simulink model "model_23b"  (R2023b)
settings: Solver=ode45  StartTime=TSPAN(1)  StopTime=TSPAN(2)  MaxStep=MaxStep  RelTol=RelTol  AbsTol=AbsTol
values from neighbouring files (symbols this model uses):
  cal_V0_ini = 0    [init.m]
  dim_xp = numel(xp_0)    [init.m]
  JSPAN = [0 30*TSPAN(2)]    [init.m]
  parameters = struct()    [init.m]
  TSPAN = [0 300]    [init.m]
  xc_0 = [chi_0;theta_0]    [init.m]
  xp_0 = [p_0;q_0;v_0;o_0]    [init.m]
libraries: HyEQ_Library x6
(part 1 of 2)
settings Model: Creator=score  LastModifiedBy=zxz
settings DataIOCC: SaveFormat=Array  ReturnWorkspaceOutputs=off

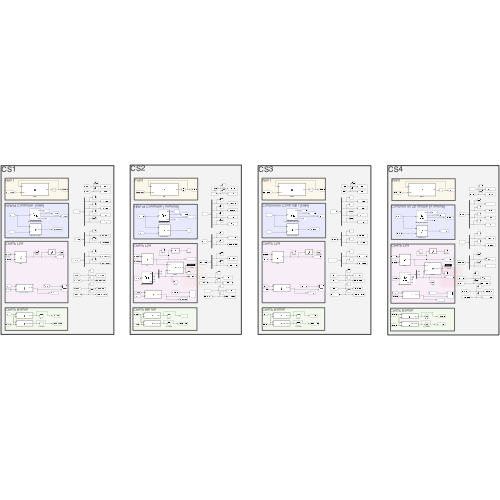
[thumbnail: Simulink's stored preview of the top-level diagram]
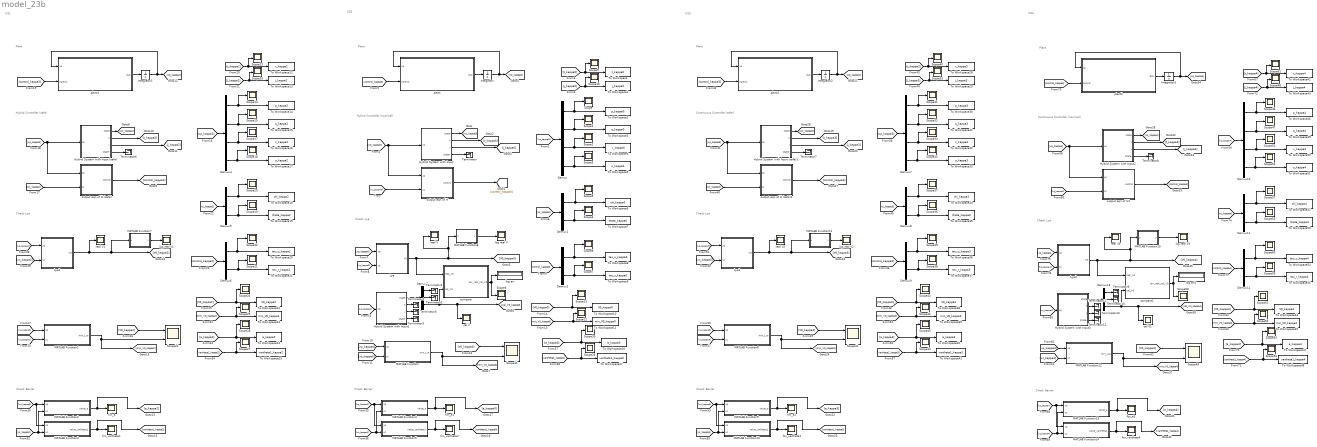
== system model_23b ==
  note: CS2
  note: CS1
  note: Check Barrier
  note: Check Lya
  note: Plant
  note: Hybrid Controller (nominal)
  note: Plant
  note: Hybrid Controller (safe)
  note: Check Lya
  note: Check Barrier
  note: CS3
  note: Continuous Controller (safe)
  note: Check Barrier
  note: Check Lya
  note: Plant
  note: CS4
  note: Check Barrier
  note: Plant
  note: Continuous Controller (nominal)
  note: Check Lya
  Demux{,4,7,10} (4 alike) : Demux  Outputs=[2;2;2;1]
  Demux{1,5,8,11} (4 alike) : Demux  Outputs=[2;1]
  Demux{2,6,9,12} (4 alike) : Demux  Outputs=[1;1]
  Demux13 : Demux  Outputs=[2;1;1]
  Demux3 : Demux  Outputs=[2;1;1]
  Hybrid System with Input : Subsystem  LoadFcn=set_param(gcb,'LinkStatus','none')  mask(Hybrid System with Inputs){x0=xc_0, input_dim=dim_xp, parameters=parameters, T=TSPAN(2), J=JSPAN(2), rule=Flow}
      mask prompts: x0 "Initial Condition (column vector)"; input_dim "Input Dimension (positive integer)"; T "Flow Horizon (nonnegative real)"; J "Jump Horizon (nonnegative integer)"; rule "Flow/Jump Priorty Rule"
      mask help:
      | To modify (f, g, C, D) for this block, "Look inside" the block mask by either clicking the down arrow in the lower-left corner or selecting "Mask" > "Look Under Mask" from the context menu.
      |
      | For instructions how to use this block, see the
      mask init:
      | state_dim = numel(x0);
      settings: CopyFcn=|
      | set_param(gcb,'LinkStatus','none'),
      | set_param(gcs, 'MaxStep', 'MaxStep', 'RelTol', 'RelTol','StopTime', 'T')
      mask Help:
      | To modify (f, g, C, D) for this block, "Look inside" the block mask by either clicking the down arrow in the lower-left corner or selecting "Mask" > "Look Under Mask" from the context menu.
      | 
      | The value given in the 'parameters' field is passed as the last input argument for f, g, C, and D. Any MATLAB object can be used, but we recommend using a struct. For example, in the initialization script, a parameters struct can be defined as followed.
      |   parameters = struct();
      |   parameters.A = eye(2);
      |   parameters.B = [1; 0];
      | 
      | The output "x-" is the state output delayed by one integration step. Use this output to break algebraic loops.
      mask TypeOptions x0: Integrator System/x0
      mask TypeOptions T: Integrator System/T
      mask TypeOptions J: Integrator System/J
      mask TypeOptions rule: Jump | Flow | Random
      mask DialogControl Control2 Prompt: Introduction to the HyEQ Simulink-based Library
      mask DialogControl Control2 Callback: hybrid.internal.openHelp('Help_SimulinkLibrary')
      mask DialogControl Container3 Prompt: System Configuration
      mask DialogControl Container2 Prompt: Solver Options
      mask Display:
      | image('Hcal.jpg')
      | port_label('output', 1, 'state')
      | port_label('output', 2, 't')
      | port_label('output', 3, 'j')
      | port_label('output', 4, 'state^-','texmode', 'on')
      | port_label('input', 1, 'xp')
  Hybrid System with Input (safe) : Subsystem  LoadFcn=set_param(gcb,'LinkStatus','none')  mask(Hybrid System with Inputs){x0=xc_0, input_dim=dim_xp, parameters=parameters, T=TSPAN(2), J=JSPAN(2), rule=Flow}
      mask prompts: x0 "Initial Condition (column vector)"; input_dim "Input Dimension (positive integer)"; T "Flow Horizon (nonnegative real)"; J "Jump Horizon (nonnegative integer)"; rule "Flow/Jump Priorty Rule"
      mask help:
      | To modify (f, g, C, D) for this block, "Look inside" the block mask by either clicking the down arrow in the lower-left corner or selecting "Mask" > "Look Under Mask" from the context menu.
      |
      | For instructions how to use this block, see the
      mask init:
      | state_dim = numel(x0);
      settings: CopyFcn=|
      | set_param(gcb,'LinkStatus','none'),
      | set_param(gcs, 'MaxStep', 'MaxStep', 'RelTol', 'RelTol','StopTime', 'T')
      mask Help:
      | To modify (f, g, C, D) for this block, "Look inside" the block mask by either clicking the down arrow in the lower-left corner or selecting "Mask" > "Look Under Mask" from the context menu.
      | 
      | The value given in the 'parameters' field is passed as the last input argument for f, g, C, and D. Any MATLAB object can be used, but we recommend using a struct. For example, in the initialization script, a parameters struct can be defined as followed.
      |   parameters = struct();
      |   parameters.A = eye(2);
      |   parameters.B = [1; 0];
      | 
      | The output "x-" is the state output delayed by one integration step. Use this output to break algebraic loops.
      mask TypeOptions x0: Integrator System/x0
      mask TypeOptions T: Integrator System/T
      mask TypeOptions J: Integrator System/J
      mask TypeOptions rule: Jump | Flow | Random
      mask DialogControl Control2 Prompt: Introduction to the HyEQ Simulink-based Library
      mask DialogControl Control2 Callback: hybrid.internal.openHelp('Help_SimulinkLibrary')
      mask DialogControl Container3 Prompt: System Configuration
      mask DialogControl Container2 Prompt: Solver Options
      mask Display:
      | image('Hcal.jpg')
      | port_label('output', 1, 'state')
      | port_label('output', 2, 't')
      | port_label('output', 3, 'j')
      | port_label('output', 4, 'state^-','texmode', 'on')
      | port_label('input', 1, 'xp')
  Hybrid System with Input (safe)1 : Subsystem  LoadFcn=set_param(gcb,'LinkStatus','none')  mask(Hybrid System with Inputs){x0=xc_0, input_dim=dim_xp, parameters=parameters, T=TSPAN(2), J=JSPAN(2), rule=Flow}
      mask prompts: x0 "Initial Condition (column vector)"; input_dim "Input Dimension (positive integer)"; T "Flow Horizon (nonnegative real)"; J "Jump Horizon (nonnegative integer)"; rule "Flow/Jump Priorty Rule"
      mask help:
      | To modify (f, g, C, D) for this block, "Look inside" the block mask by either clicking the down arrow in the lower-left corner or selecting "Mask" > "Look Under Mask" from the context menu.
      |
      | For instructions how to use this block, see the
      mask init:
      | state_dim = numel(x0);
      settings: CopyFcn=|
      | set_param(gcb,'LinkStatus','none'),
      | set_param(gcs, 'MaxStep', 'MaxStep', 'RelTol', 'RelTol','StopTime', 'T')
      mask Help:
      | To modify (f, g, C, D) for this block, "Look inside" the block mask by either clicking the down arrow in the lower-left corner or selecting "Mask" > "Look Under Mask" from the context menu.
      | 
      | The value given in the 'parameters' field is passed as the last input argument for f, g, C, and D. Any MATLAB object can be used, but we recommend using a struct. For example, in the initialization script, a parameters struct can be defined as followed.
      |   parameters = struct();
      |   parameters.A = eye(2);
      |   parameters.B = [1; 0];
      | 
      | The output "x-" is the state output delayed by one integration step. Use this output to break algebraic loops.
      mask TypeOptions x0: Integrator System/x0
      mask TypeOptions T: Integrator System/T
      mask TypeOptions J: Integrator System/J
      mask TypeOptions rule: Jump | Flow | Random
      mask DialogControl Control2 Prompt: Introduction to the HyEQ Simulink-based Library
      mask DialogControl Control2 Callback: hybrid.internal.openHelp('Help_SimulinkLibrary')
      mask DialogControl Container3 Prompt: System Configuration
      mask DialogControl Container2 Prompt: Solver Options
      mask Display:
      | image('Hcal.jpg')
      | port_label('output', 1, 'state')
      | port_label('output', 2, 't')
      | port_label('output', 3, 'j')
      | port_label('output', 4, 'state^-','texmode', 'on')
      | port_label('input', 1, 'xp')
  Hybrid System with Input1 : Subsystem  LoadFcn=set_param(gcb,'LinkStatus','none')  mask(Hybrid System with Inputs){x0=[xc_0;cal_V0_ini], input_dim=dim_xp, parameters=parameters, T=TSPAN(2), J=JSPAN(2), rule=Flow}
      mask prompts: x0 "Initial Condition (column vector)"; input_dim "Input Dimension (positive integer)"; T "Flow Horizon (nonnegative real)"; J "Jump Horizon (nonnegative integer)"; rule "Flow/Jump Priorty Rule"
      mask help:
      | To modify (f, g, C, D) for this block, "Look inside" the block mask by either clicking the down arrow in the lower-left corner or selecting "Mask" > "Look Under Mask" from the context menu.
      |
      | For instructions how to use this block, see the
      mask init:
      | state_dim = numel(x0);
      settings: CopyFcn=|
      | set_param(gcb,'LinkStatus','none'),
      | set_param(gcs, 'MaxStep', 'MaxStep', 'RelTol', 'RelTol','StopTime', 'T')
      mask Help:
      | To modify (f, g, C, D) for this block, "Look inside" the block mask by either clicking the down arrow in the lower-left corner or selecting "Mask" > "Look Under Mask" from the context menu.
      | 
      | The value given in the 'parameters' field is passed as the last input argument for f, g, C, and D. Any MATLAB object can be used, but we recommend using a struct. For example, in the initialization script, a parameters struct can be defined as followed.
      |   parameters = struct();
      |   parameters.A = eye(2);
      |   parameters.B = [1; 0];
      | 
      | The output "x-" is the state output delayed by one integration step. Use this output to break algebraic loops.
      mask TypeOptions x0: Integrator System/x0
      mask TypeOptions T: Integrator System/T
      mask TypeOptions J: Integrator System/J
      mask TypeOptions rule: Jump | Flow | Random
      mask DialogControl Control2 Prompt: Introduction to the HyEQ Simulink-based Library
      mask DialogControl Control2 Callback: hybrid.internal.openHelp('Help_SimulinkLibrary')
      mask DialogControl Container3 Prompt: System Configuration
      mask DialogControl Container2 Prompt: Solver Options
      mask Display:
      | image('Hcal.jpg')
      | port_label('output', 1, 'state')
      | port_label('output', 2, 't')
      | port_label('output', 3, 'j')
      | port_label('output', 4, 'state^-','texmode', 'on')
      | port_label('input', 1, 'xp')
  Hybrid System with Input2 : Subsystem  LoadFcn=set_param(gcb,'LinkStatus','none')  mask(Hybrid System with Inputs){x0=xc_0, input_dim=dim_xp, parameters=parameters, T=TSPAN(2), J=JSPAN(2), rule=Flow}
      mask prompts: x0 "Initial Condition (column vector)"; input_dim "Input Dimension (positive integer)"; T "Flow Horizon (nonnegative real)"; J "Jump Horizon (nonnegative integer)"; rule "Flow/Jump Priorty Rule"
      mask help:
      | To modify (f, g, C, D) for this block, "Look inside" the block mask by either clicking the down arrow in the lower-left corner or selecting "Mask" > "Look Under Mask" from the context menu.
      |
      | For instructions how to use this block, see the
      mask init:
      | state_dim = numel(x0);
      settings: CopyFcn=|
      | set_param(gcb,'LinkStatus','none'),
      | set_param(gcs, 'MaxStep', 'MaxStep', 'RelTol', 'RelTol','StopTime', 'T')
      mask Help:
      | To modify (f, g, C, D) for this block, "Look inside" the block mask by either clicking the down arrow in the lower-left corner or selecting "Mask" > "Look Under Mask" from the context menu.
      | 
      | The value given in the 'parameters' field is passed as the last input argument for f, g, C, and D. Any MATLAB object can be used, but we recommend using a struct. For example, in the initialization script, a parameters struct can be defined as followed.
      |   parameters = struct();
      |   parameters.A = eye(2);
      |   parameters.B = [1; 0];
      | 
      | The output "x-" is the state output delayed by one integration step. Use this output to break algebraic loops.
      mask TypeOptions x0: Integrator System/x0
      mask TypeOptions T: Integrator System/T
      mask TypeOptions J: Integrator System/J
      mask TypeOptions rule: Jump | Flow | Random
      mask DialogControl Control2 Prompt: Introduction to the HyEQ Simulink-based Library
      mask DialogControl Control2 Callback: hybrid.internal.openHelp('Help_SimulinkLibrary')
      mask DialogControl Container3 Prompt: System Configuration
      mask DialogControl Container2 Prompt: Solver Options
      mask Display:
      | image('Hcal.jpg')
      | port_label('output', 1, 'state')
      | port_label('output', 2, 't')
      | port_label('output', 3, 'j')
      | port_label('output', 4, 'state^-','texmode', 'on')
      | port_label('input', 1, 'xp')
  Hybrid System with Input3 : Subsystem  LoadFcn=set_param(gcb,'LinkStatus','none')  mask(Hybrid System with Inputs){x0=[xc_0;cal_V0_ini], input_dim=dim_xp, parameters=parameters, T=TSPAN(2), J=JSPAN(2), rule=Flow}
      mask prompts: x0 "Initial Condition (column vector)"; input_dim "Input Dimension (positive integer)"; T "Flow Horizon (nonnegative real)"; J "Jump Horizon (nonnegative integer)"; rule "Flow/Jump Priorty Rule"
      mask help:
      | To modify (f, g, C, D) for this block, "Look inside" the block mask by either clicking the down arrow in the lower-left corner or selecting "Mask" > "Look Under Mask" from the context menu.
      |
      | For instructions how to use this block, see the
      mask init:
      | state_dim = numel(x0);
      settings: CopyFcn=|
      | set_param(gcb,'LinkStatus','none'),
      | set_param(gcs, 'MaxStep', 'MaxStep', 'RelTol', 'RelTol','StopTime', 'T')
      mask Help:
      | To modify (f, g, C, D) for this block, "Look inside" the block mask by either clicking the down arrow in the lower-left corner or selecting "Mask" > "Look Under Mask" from the context menu.
      | 
      | The value given in the 'parameters' field is passed as the last input argument for f, g, C, and D. Any MATLAB object can be used, but we recommend using a struct. For example, in the initialization script, a parameters struct can be defined as followed.
      |   parameters = struct();
      |   parameters.A = eye(2);
      |   parameters.B = [1; 0];
      | 
      | The output "x-" is the state output delayed by one integration step. Use this output to break algebraic loops.
      mask TypeOptions x0: Integrator System/x0
      mask TypeOptions T: Integrator System/T
      mask TypeOptions J: Integrator System/J
      mask TypeOptions rule: Jump | Flow | Random
      mask DialogControl Control2 Prompt: Introduction to the HyEQ Simulink-based Library
      mask DialogControl Control2 Callback: hybrid.internal.openHelp('Help_SimulinkLibrary')
      mask DialogControl Container3 Prompt: System Configuration
      mask DialogControl Container2 Prompt: Solver Options
      mask Display:
      | image('Hcal.jpg')
      | port_label('output', 1, 'state')
      | port_label('output', 2, 't')
      | port_label('output', 3, 'j')
      | port_label('output', 4, 'state^-','texmode', 'on')
      | port_label('input', 1, 'xp')
  Integrator{,1..3} (4 alike) : Integrator  InitialCondition=xp_0
  Lya : MATLAB Function  TreatAsAtomicUnit=on
  Lya1 : MATLAB Function  TreatAsAtomicUnit=on
  Lya2 : MATLAB Function  TreatAsAtomicUnit=on
  Lya3 : MATLAB Function  TreatAsAtomicUnit=on
  MATLAB Function : MATLAB Function  TreatAsAtomicUnit=on
  MATLAB Function1 : MATLAB Function  TreatAsAtomicUnit=on
  MATLAB Function10 : MATLAB Function  TreatAsAtomicUnit=on
  MATLAB Function11 : MATLAB Function  TreatAsAtomicUnit=on
  MATLAB Function12 : MATLAB Function  TreatAsAtomicUnit=on
  MATLAB Function13 : MATLAB Function  TreatAsAtomicUnit=on
  MATLAB Function14 : MATLAB Function  TreatAsAtomicUnit=on
  MATLAB Function15 : MATLAB Function  TreatAsAtomicUnit=on
  MATLAB Function2 : MATLAB Function  TreatAsAtomicUnit=on
  MATLAB Function3 : MATLAB Function  TreatAsAtomicUnit=on
  MATLAB Function4 : MATLAB Function  TreatAsAtomicUnit=on
  MATLAB Function5 : MATLAB Function  TreatAsAtomicUnit=on
  MATLAB Function6 : MATLAB Function  TreatAsAtomicUnit=on
  MATLAB Function7 : MATLAB Function  TreatAsAtomicUnit=on
  MATLAB Function8 : MATLAB Function  TreatAsAtomicUnit=on
  MATLAB Function9 : MATLAB Function  TreatAsAtomicUnit=on
  Scope{,1..10,12..23,25..40,42..48,50..61} (58 alike) : Scope
  Scope{11,24,41,49} (4 alike) : Scope  NumInputPorts=2
  Terminator{,1..13} (14 alike) : Terminator
  To Workspace : ToWorkspace  VariableName=t_kappa0  SaveFormat=Structure  SampleTime=-1
      settings: Save2DSignal=2-D array (concatenate along first dimension)
  To Workspace1 : ToWorkspace  VariableName=j_kappa0  SaveFormat=Structure  SampleTime=-1
      settings: Save2DSignal=2-D array (concatenate along first dimension)
  To Workspace10 : ToWorkspace  VariableName=V0_kappa0  SaveFormat=Structure  SampleTime=-1
      settings: Save2DSignal=2-D array (concatenate along first dimension)
  To Workspace11 : ToWorkspace  VariableName=min_V0_kappa0  SaveFormat=Structure  SampleTime=-1
      settings: Save2DSignal=2-D array (concatenate along first dimension)
  To Workspace12 : ToWorkspace  VariableName=t_kappa2  SaveFormat=Structure  SampleTime=-1
      settings: Save2DSignal=2-D array (concatenate along first dimension)
  To Workspace13 : ToWorkspace  VariableName=j_kappa2  SaveFormat=Structure  SampleTime=-1
      settings: Save2DSignal=2-D array (concatenate along first dimension)
  To Workspace14 : ToWorkspace  VariableName=p_kappa2  SaveFormat=Structure  SampleTime=-1
      settings: Save2DSignal=2-D array (concatenate along first dimension)
  To Workspace15 : ToWorkspace  VariableName=q_kappa2  SaveFormat=Structure  SampleTime=-1
      settings: Save2DSignal=2-D array (concatenate along first dimension)
  To Workspace16 : ToWorkspace  VariableName=v_kappa2  SaveFormat=Structure  SampleTime=-1
      settings: Save2DSignal=2-D array (concatenate along first dimension)
  To Workspace17 : ToWorkspace  VariableName=o_kappa2  SaveFormat=Structure  SampleTime=-1
      settings: Save2DSignal=2-D array (concatenate along first dimension)
  To Workspace18 : ToWorkspace  VariableName=chi_kappa2  SaveFormat=Structure  SampleTime=-1
      settings: Save2DSignal=2-D array (concatenate along first dimension)
  To Workspace19 : ToWorkspace  VariableName=theta_kappa2  SaveFormat=Structure  SampleTime=-1
      settings: Save2DSignal=2-D array (concatenate along first dimension)
  To Workspace2 : ToWorkspace  VariableName=p_kappa0  SaveFormat=Structure  SampleTime=-1
      settings: Save2DSignal=2-D array (concatenate along first dimension)
  To Workspace20 : ToWorkspace  VariableName=tau_u_kappa2  SaveFormat=Structure  SampleTime=-1
      settings: Save2DSignal=2-D array (concatenate along first dimension)
  To Workspace21 : ToWorkspace  VariableName=tau_r_kappa2  SaveFormat=Structure  SampleTime=-1
      settings: Save2DSignal=2-D array (concatenate along first dimension)
  To Workspace22 : ToWorkspace  VariableName=V0_kappa2  SaveFormat=Structure  SampleTime=-1
      settings: Save2DSignal=2-D array (concatenate along first dimension)
  To Workspace23 : ToWorkspace  VariableName=min_V0_kappa2  SaveFormat=Structure  SampleTime=-1
      settings: Save2DSignal=2-D array (concatenate along first dimension)
  To Workspace24 : ToWorkspace  VariableName=a_kappa2  SaveFormat=Structure  SampleTime=-1
      settings: Save2DSignal=2-D array (concatenate along first dimension)
  To Workspace25 : ToWorkspace  VariableName=vartheta1_kappa2  SaveFormat=Structure  SampleTime=-1
      settings: Save2DSignal=2-D array (concatenate along first dimension)
  To Workspace26 : ToWorkspace  VariableName=a_kappa0  SaveFormat=Structure  SampleTime=-1
      settings: Save2DSignal=2-D array (concatenate along first dimension)
  To Workspace27 : ToWorkspace  VariableName=vartheta1_kappa0  SaveFormat=Structure  SampleTime=-1
      settings: Save2DSignal=2-D array (concatenate along first dimension)
  To Workspace28 : ToWorkspace  VariableName=t_kappa3  SaveFormat=Structure  SampleTime=-1
      settings: Save2DSignal=2-D array (concatenate along first dimension)
  To Workspace29 : ToWorkspace  VariableName=j_kappa3  SaveFormat=Structure  SampleTime=-1
      settings: Save2DSignal=2-D array (concatenate along first dimension)
  To Workspace3 : ToWorkspace  VariableName=q_kappa0  SaveFormat=Structure  SampleTime=-1
      settings: Save2DSignal=2-D array (concatenate along first dimension)
  To Workspace30 : ToWorkspace  VariableName=p_kappa3  SaveFormat=Structure  SampleTime=-1
      settings: Save2DSignal=2-D array (concatenate along first dimension)
  To Workspace31 : ToWorkspace  VariableName=q_kappa3  SaveFormat=Structure  SampleTime=-1
      settings: Save2DSignal=2-D array (concatenate along first dimension)
  To Workspace32 : ToWorkspace  VariableName=v_kappa3  SaveFormat=Structure  SampleTime=-1
      settings: Save2DSignal=2-D array (concatenate along first dimension)
  To Workspace33 : ToWorkspace  VariableName=o_kappa3  SaveFormat=Structure  SampleTime=-1
      settings: Save2DSignal=2-D array (concatenate along first dimension)
  To Workspace34 : ToWorkspace  VariableName=chi_kappa3  SaveFormat=Structure  SampleTime=-1
      settings: Save2DSignal=2-D array (concatenate along first dimension)
  To Workspace35 : ToWorkspace  VariableName=theta_kappa3  SaveFormat=Structure  SampleTime=-1
      settings: Save2DSignal=2-D array (concatenate along first dimension)
  To Workspace36 : ToWorkspace  VariableName=tau_u_kappa3  SaveFormat=Structure  SampleTime=-1
      settings: Save2DSignal=2-D array (concatenate along first dimension)
  To Workspace37 : ToWorkspace  VariableName=tau_r_kappa3  SaveFormat=Structure  SampleTime=-1
      settings: Save2DSignal=2-D array (concatenate along first dimension)
  To Workspace38 : ToWorkspace  VariableName=V0_kappa3  SaveFormat=Structure  SampleTime=-1
      settings: Save2DSignal=2-D array (concatenate along first dimension)
  To Workspace39 : ToWorkspace  VariableName=min_V0_kappa3  SaveFormat=Structure  SampleTime=-1
      settings: Save2DSignal=2-D array (concatenate along first dimension)
  To Workspace4 : ToWorkspace  VariableName=v_kappa0  SaveFormat=Structure  SampleTime=-1
      settings: Save2DSignal=2-D array (concatenate along first dimension)
  To Workspace40 : ToWorkspace  VariableName=a_kappa3  SaveFormat=Structure  SampleTime=-1
      settings: Save2DSignal=2-D array (concatenate along first dimension)
  To Workspace41 : ToWorkspace  VariableName=vartheta1_kappa3  SaveFormat=Structure  SampleTime=-1
      settings: Save2DSignal=2-D array (concatenate along first dimension)
  To Workspace42 : ToWorkspace  VariableName=t_kappa4  SaveFormat=Structure  SampleTime=-1
      settings: Save2DSignal=2-D array (concatenate along first dimension)
  To Workspace43 : ToWorkspace  VariableName=j_kappa4  SaveFormat=Structure  SampleTime=-1
      settings: Save2DSignal=2-D array (concatenate along first dimension)
  To Workspace44 : ToWorkspace  VariableName=V0_kappa4  SaveFormat=Structure  SampleTime=-1
      settings: Save2DSignal=2-D array (concatenate along first dimension)
  To Workspace45 : ToWorkspace  VariableName=min_V0_kappa4  SaveFormat=Structure  SampleTime=-1
      settings: Save2DSignal=2-D array (concatenate along first dimension)
  To Workspace46 : ToWorkspace  VariableName=p_kappa4  SaveFormat=Structure  SampleTime=-1
      settings: Save2DSignal=2-D array (concatenate along first dimension)
  To Workspace47 : ToWorkspace  VariableName=a_kappa4  SaveFormat=Structure  SampleTime=-1
      settings: Save2DSignal=2-D array (concatenate along first dimension)
  To Workspace48 : ToWorkspace  VariableName=vartheta1_kappa4  SaveFormat=Structure  SampleTime=-1
      settings: Save2DSignal=2-D array (concatenate along first dimension)
  To Workspace49 : ToWorkspace  VariableName=q_kappa4  SaveFormat=Structure  SampleTime=-1
      settings: Save2DSignal=2-D array (concatenate along first dimension)
  To Workspace5 : ToWorkspace  VariableName=o_kappa0  SaveFormat=Structure  SampleTime=-1
      settings: Save2DSignal=2-D array (concatenate along first dimension)
  To Workspace50 : ToWorkspace  VariableName=v_kappa4  SaveFormat=Structure  SampleTime=-1
      settings: Save2DSignal=2-D array (concatenate along first dimension)
  To Workspace51 : ToWorkspace  VariableName=o_kappa4  SaveFormat=Structure  SampleTime=-1
      settings: Save2DSignal=2-D array (concatenate along first dimension)
  To Workspace52 : ToWorkspace  VariableName=chi_kappa4  SaveFormat=Structure  SampleTime=-1
      settings: Save2DSignal=2-D array (concatenate along first dimension)
  To Workspace53 : ToWorkspace  VariableName=theta_kappa4  SaveFormat=Structure  SampleTime=-1
      settings: Save2DSignal=2-D array (concatenate along first dimension)
  To Workspace54 : ToWorkspace  VariableName=tau_u_kappa4  SaveFormat=Structure  SampleTime=-1
      settings: Save2DSignal=2-D array (concatenate along first dimension)
  To Workspace55 : ToWorkspace  VariableName=tau_r_kappa4  SaveFormat=Structure  SampleTime=-1
      settings: Save2DSignal=2-D array (concatenate along first dimension)
  To Workspace6 : ToWorkspace  VariableName=chi_kappa0  SaveFormat=Structure  SampleTime=-1
      settings: Save2DSignal=2-D array (concatenate along first dimension)
  To Workspace7 : ToWorkspace  VariableName=theta_kappa0  SaveFormat=Structure  SampleTime=-1
      settings: Save2DSignal=2-D array (concatenate along first dimension)
  To Workspace8 : ToWorkspace  VariableName=tau_u_kappa0  SaveFormat=Structure  SampleTime=-1
      settings: Save2DSignal=2-D array (concatenate along first dimension)
  To Workspace9 : ToWorkspace  VariableName=tau_r_kappa0  SaveFormat=Structure  SampleTime=-1
      settings: Save2DSignal=2-D array (concatenate along first dimension)
  cal V : Scope
  cal V1 : Scope
  compare : MATLAB Function  TreatAsAtomicUnit=on
  compare1 : MATLAB Function  TreatAsAtomicUnit=on
  fcn_a{,1..3} (4 alike) : Scope
  fcn_vartheta{1..4} (4 alike) : Scope
  log err : Display
  log err1 : Display
  log real V{,1..3} (4 alike) : Scope
  output eqn of H : MATLAB Function  TreatAsAtomicUnit=on
  output eqn of H (safe) : MATLAB Function  TreatAsAtomicUnit=on
  output eqn of H (safe)1 : MATLAB Function  TreatAsAtomicUnit=on
  output eqn of H1 : MATLAB Function  TreatAsAtomicUnit=on
  plant : MATLAB Function  TreatAsAtomicUnit=on
  plant1 : MATLAB Function  TreatAsAtomicUnit=on
  plant2 : MATLAB Function  TreatAsAtomicUnit=on
  plant3 : MATLAB Function  TreatAsAtomicUnit=on
  real V{,1..3} (4 alike) : Scope
  wires:
  Hybrid System with Input/4(state-) -> Terminator/1
  Hybrid System with Input/2(t) -> [t_kappa0]
  Hybrid System with Input/3(j) -> [j_kappa0]
  Hybrid System with Input/1(state) -> [xc_kappa0]
  [xp_kappa0] -> output eqn of H/1(xp), Hybrid System with Input/1(xp)
  [xc_kappa0] -> output eqn of H/2(xc)
  output eqn of H/1(control) -> [control_kappa0]
  [t_kappa0] -> Scope9/1, To Workspace/1
  [j_kappa0] -> Scope10/1, To Workspace1/1
  plant/1(dxp) -> Integrator/1
  [control_kappa0] -> plant/2(control)
  Integrator/1 -> plant/1(xp), [xp_kappa0]
  [xp_kappa0] -> Demux/1
  [xc_kappa0] -> Demux1/1
  Demux/1 -> Scope/1, To Workspace2/1
  Demux/2 -> Scope1/1, To Workspace3/1
  Demux/3 -> Scope2/1, To Workspace4/1
  Demux/4 -> Scope3/1, To Workspace5/1
  Demux1/2 -> Scope4/1, To Workspace7/1
  Demux1/1 -> Scope5/1, To Workspace6/1
  [xp_kappa0] -> Lya/1(xp)
  [xc_kappa0] -> Lya/2(xc)
  compare/1(err_real_cal_V0) -> Scope6/1, log err/1
  Lya/1(V0) -> compare/1(real_V0), [V0_kappa0], MATLAB Function6/1(u), real V/1
  [control_kappa0] -> Demux2/1
  Demux2/2 -> Scope7/1, To Workspace9/1
  Demux2/1 -> To Workspace8/1, Scope8/1
  [xp_kappa0] -> MATLAB Function/1(xp)
  [xc_kappa0] -> MATLAB Function/2(xc)
  Hybrid System with Input1/3(j) -> Terminator5/1
  Hybrid System with Input1/2(t) -> Terminator4/1
  Hybrid System with Input1/1(state) -> Demux3/1
  [xp_kappa0] -> Hybrid System with Input1/1(xp)
  Hybrid System with Input1/4(state-) -> Terminator3/1
  Demux3/1 -> Terminator1/1
  Demux3/2 -> Terminator2/1
  Demux3/3 -> [cal_V0_kappa0], cal V/1, compare/2(cal_V0)
  MATLAB Function/1(min_Lya) -> Scope11/2, [min_V0_kappa0]
  [V0_kappa0] -> Scope11/1
  [V0_kappa0] -> Scope13/1, To Workspace10/1
  [min_V0_kappa0] -> Scope12/1, To Workspace11/1
  output eqn of H (safe)/1(control) -> [control_kappa2]
  Hybrid System with Input (safe)/3(j) -> [j_kappa2]
  [xc_kappa2] -> output eqn of H (safe)/2(xc)
  [control_kappa2] -> plant1/2(control)
  Hybrid System with Input (safe)/2(t) -> [t_kappa2]
  Hybrid System with Input (safe)/1(state) -> [xc_kappa2]
  [xp_kappa2] -> output eqn of H (safe)/1(xp), Hybrid System with Input (safe)/1(xp)
  plant1/1(dxp) -> Integrator1/1
  Hybrid System with Input (safe)/4(state-) -> Terminator6/1
  Integrator1/1 -> plant1/1(xp), [xp_kappa2]
  Demux5/2 -> Scope19/1, To Workspace19/1
  [xc_kappa2] -> Demux5/1
  [t_kappa2] -> Scope23/1, To Workspace12/1
  [control_kappa2] -> Demux6/1
  Demux5/1 -> Scope20/1, To Workspace18/1
  Demux4/1 -> Scope14/1, To Workspace14/1
  [xp_kappa2] -> Demux4/1
  Demux4/2 -> Scope15/1, To Workspace15/1
  Demux4/3 -> Scope17/1, To Workspace16/1
  Demux4/4 -> Scope18/1, To Workspace17/1
  [j_kappa2] -> Scope16/1, To Workspace13/1
  Demux6/1 -> To Workspace20/1, Scope22/1
  Demux6/2 -> Scope21/1, To Workspace21/1
  MATLAB Function1/1(min_Lya) -> Scope24/2, [min_V0_kappa2]
  [xp_kappa2] -> MATLAB Function1/1(xp)
  [xc_kappa2] -> Lya2/2(xc)
  [xp_kappa2] -> Lya2/1(xp)
  [V0_kappa2] -> Scope24/1
  [xc_kappa2] -> MATLAB Function1/2(xc)
  [min_V0_kappa2] -> Scope25/1, To Workspace23/1
  [V0_kappa2] -> Scope26/1, To Workspace22/1
  [xp_kappa2] -> MATLAB Function3/1(xp), MATLAB Function2/1(xp)
  [xc_kappa2] -> MATLAB Function2/2(xc), MATLAB Function3/2(xc)
  MATLAB Function3/1(value_vartheta1) -> [vartheta1_kappa2], fcn_vartheta1/1
  MATLAB Function2/1(value_a) -> [a_kappa2], fcn_a/1
  [vartheta1_kappa2] -> Scope27/1, To Workspace25/1
  [a_kappa2] -> Scope28/1, To Workspace24/1
  [xp_kappa0] -> MATLAB Function5/1(xp), MATLAB Function4/1(xp)
  MATLAB Function4/1(value_a) -> [a_kappa0], fcn_a1/1
  [xc_kappa0] -> MATLAB Function4/2(xc), MATLAB Function5/2(xc)
  MATLAB Function5/1(value_vartheta1) -> [vartheta1_kappa0], fcn_vartheta2/1
  [vartheta1_kappa0] -> Scope29/1, To Workspace27/1
  [a_kappa0] -> Scope30/1, To Workspace26/1
  MATLAB Function6/1(y) -> log real V/1
  Lya2/1(V0) -> MATLAB Function7/1(u), [V0_kappa2], real V1/1
  MATLAB Function7/1(y) -> log real V1/1
  [xp_kappa3] -> Demux7/1
  [xp_kappa3] -> MATLAB Function10/1(xp), MATLAB Function9/1(xp)
  [t_kappa3] -> Scope40/1, To Workspace28/1
  [xc_kappa3] -> MATLAB Function9/2(xc), MATLAB Function10/2(xc)
  [V0_kappa3] -> Scope41/1
  MATLAB Function9/1(value_a) -> [a_kappa3], fcn_a2/1
  output eqn of H (safe)1/1(control) -> [control_kappa3]
  [xc_kappa3] -> MATLAB Function8/2(xc)
  MATLAB Function10/1(value_vartheta1) -> [vartheta1_kappa3], fcn_vartheta3/1
  [xp_kappa3] -> Lya1/1(xp)
  [control_kappa3] -> Demux9/1
  [xp_kappa3] -> MATLAB Function8/1(xp)
  Hybrid System with Input (safe)1/1(state) -> [xc_kappa3]
  Hybrid System with Input (safe)1/3(j) -> [j_kappa3]
  Demux7/1 -> Scope31/1, To Workspace30/1
  Demux8/2 -> Scope36/1, To Workspace35/1
  plant2/1(dxp) -> Integrator2/1
  MATLAB Function8/1(min_Lya) -> Scope41/2, [min_V0_kappa3]
  Hybrid System with Input (safe)1/2(t) -> [t_kappa3]
  Lya1/1(V0) -> MATLAB Function11/1(u), [V0_kappa3], real V2/1
  [V0_kappa3] -> Scope43/1, To Workspace38/1
  Demux7/4 -> Scope35/1, To Workspace33/1
  [a_kappa3] -> Scope45/1, To Workspace40/1
  [xc_kappa3] -> Lya1/2(xc)
  Integrator2/1 -> plant2/1(xp), [xp_kappa3]
  [vartheta1_kappa3] -> Scope44/1, To Workspace41/1
  MATLAB Function11/1(y) -> log real V2/1
  [control_kappa3] -> plant2/2(control)
  Demux9/1 -> To Workspace36/1, Scope39/1
  [min_V0_kappa3] -> Scope42/1, To Workspace39/1
  [xp_kappa3] -> output eqn of H (safe)1/1(xp), Hybrid System with Input (safe)1/1(xp)
  Demux7/2 -> Scope32/1, To Workspace31/1
  Hybrid System with Input (safe)1/4(state-) -> Terminator7/1
  [j_kappa3] -> Scope33/1, To Workspace29/1
  Demux9/2 -> Scope38/1, To Workspace37/1
  Demux7/3 -> Scope34/1, To Workspace32/1
  [xc_kappa3] -> output eqn of H (safe)1/2(xc)
  Demux8/1 -> Scope37/1, To Workspace34/1
  [xc_kappa3] -> Demux8/1
  Demux10/2 -> Scope47/1, To Workspace49/1
  [vartheta1_kappa4] -> Scope53/1, To Workspace48/1
  [control_kappa4] -> Demux12/1
  Demux12/2 -> Scope59/1, To Workspace55/1
  [t_kappa4] -> Scope61/1, To Workspace42/1
  [j_kappa4] -> Scope48/1, To Workspace43/1
  [xc_kappa4] -> MATLAB Function13/2(xc), MATLAB Function14/2(xc)
  MATLAB Function15/1(y) -> log real V3/1
  Hybrid System with Input2/1(state) -> [xc_kappa4]
  Hybrid System with Input3/1(state) -> Demux13/1
  [xc_kappa4] -> output eqn of H1/2(xc)
  Demux13/2 -> Terminator10/1
  Demux10/1 -> Scope46/1, To Workspace46/1
  Lya3/1(V0) -> compare1/1(real_V0), [V0_kappa4], MATLAB Function15/1(u), real V3/1
  Hybrid System with Input3/4(state-) -> Terminator11/1
  Demux11/1 -> Scope57/1, To Workspace52/1
  MATLAB Function13/1(value_a) -> [a_kappa4], fcn_a3/1
  Demux10/4 -> Scope54/1, To Workspace51/1
  compare1/1(err_real_cal_V0) -> Scope58/1, log err1/1
  Demux13/1 -> Terminator9/1
  Demux10/3 -> Scope52/1, To Workspace50/1
  Hybrid System with Input3/2(t) -> Terminator12/1
  MATLAB Function14/1(value_vartheta1) -> [vartheta1_kappa4], fcn_vartheta4/1
  [xp_kappa4] -> MATLAB Function12/1(xp)
  [a_kappa4] -> Scope55/1, To Workspace47/1
  [min_V0_kappa4] -> Scope50/1, To Workspace45/1
  Hybrid System with Input2/3(j) -> [j_kappa4]
  [xp_kappa4] -> output eqn of H1/1(xp), Hybrid System with Input2/1(xp)
  Hybrid System with Input2/4(state-) -> Terminator8/1
  MATLAB Function12/1(min_Lya) -> Scope49/2, [min_V0_kappa4]
  plant3/1(dxp) -> Integrator3/1
  Demux12/1 -> To Workspace54/1, Scope60/1
  [control_kappa4] -> plant3/2(control)
  [xc_kappa4] -> Demux11/1
  Hybrid System with Input3/3(j) -> Terminator13/1
  [V0_kappa4] -> Scope51/1, To Workspace44/1
  Integrator3/1 -> plant3/1(xp), [xp_kappa4]
  [xc_kappa4] -> Lya3/2(xc)
  output eqn of H1/1(control) -> [control_kappa4]
  [xp_kappa4] -> Hybrid System with Input3/1(xp)
  Hybrid System with Input2/2(t) -> [t_kappa4]
  Demux11/2 -> Scope56/1, To Workspace53/1
  Demux13/3 -> [cal_V0_kappa4], cal V1/1, compare1/2(cal_V0)
  [xp_kappa4] -> MATLAB Function14/1(xp), MATLAB Function13/1(xp)
  [xp_kappa4] -> Lya3/1(xp)
  [xp_kappa4] -> Demux10/1
  [V0_kappa4] -> Scope49/1
  [xc_kappa4] -> MATLAB Function12/2(xc)

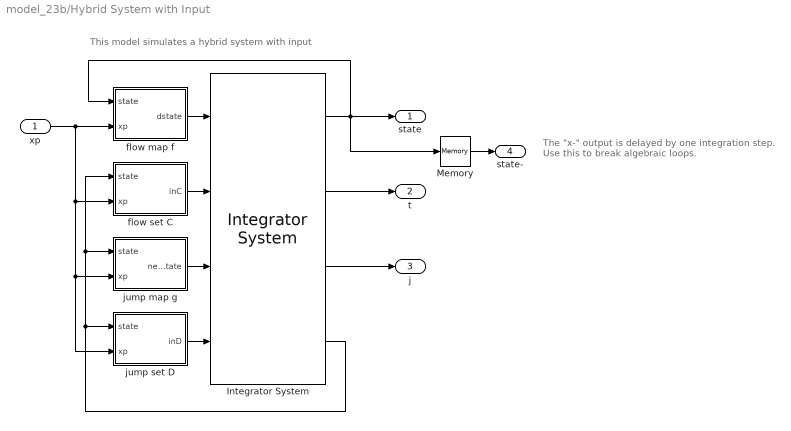
== system model_23b/Hybrid System with Input ==
  note: This model simulates a hybrid system with input
  note: The "x-" output is delayed by one integration step. Use this to break algebraic loops.
  xp : Inport  PortDimensions=input_dim
  Integrator System : HyEQ_Library/Other/Integrator System  Priority=2  T=T  J=J  x0=x0  rule=rule
      link override ICx: Value=xc_0
      link override ICx0: Value=[0; 0; xc_0(:)]
      settings: SourceProductName=Hybrid Equations Toolbox
  Memory : Memory  InitialCondition=x0
  flow map f : MATLAB Function  TreatAsAtomicUnit=on
  flow set C : MATLAB Function  TreatAsAtomicUnit=on
  jump map g : MATLAB Function  TreatAsAtomicUnit=on
  jump set D : MATLAB Function  TreatAsAtomicUnit=on
  state : Outport  PortDimensions=state_dim
  t : Outport  Port=2  PortDimensions=1
  j : Outport  Port=3  PortDimensions=1
  state- : Outport  Port=4  PortDimensions=state_dim
  wires:
  Memory/1 -> state-/1
  jump map g/1(nextstate) -> Integrator System/3
  jump set D/1(inD) -> Integrator System/4
  xp/1 -> jump set D/2(xp), jump map g/2(xp), flow set C/2(xp), flow map f/2(xp)
  Integrator System/3 -> j/1
  Integrator System/2 -> t/1
  flow set C/1(inC) -> Integrator System/2
  Integrator System/1 -> state/1, flow map f/1(state), Memory/1
  Integrator System/4 -> jump set D/1(state), jump map g/1(state), flow set C/1(state)
  flow map f/1(dstate) -> Integrator System/1

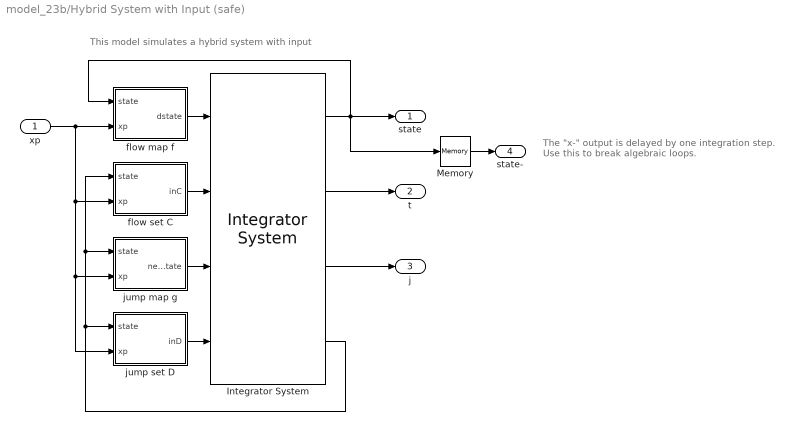
== system model_23b/Hybrid System with Input (safe) ==
  note: This model simulates a hybrid system with input
  note: The "x-" output is delayed by one integration step. Use this to break algebraic loops.
  xp : Inport  PortDimensions=input_dim
  Integrator System : HyEQ_Library/Other/Integrator System  Priority=2  T=T  J=J  x0=x0  rule=rule
      link override ICx: Value=xc_0
      link override ICx0: Value=[0; 0; xc_0(:)]
      settings: SourceProductName=Hybrid Equations Toolbox
  Memory : Memory  InitialCondition=x0
  flow map f : MATLAB Function  TreatAsAtomicUnit=on
  flow set C : MATLAB Function  TreatAsAtomicUnit=on
  jump map g : MATLAB Function  TreatAsAtomicUnit=on
  jump set D : MATLAB Function  TreatAsAtomicUnit=on
  state : Outport  PortDimensions=state_dim
  t : Outport  Port=2  PortDimensions=1
  j : Outport  Port=3  PortDimensions=1
  state- : Outport  Port=4  PortDimensions=state_dim
  wires:
  Memory/1 -> state-/1
  jump map g/1(nextstate) -> Integrator System/3
  jump set D/1(inD) -> Integrator System/4
  xp/1 -> jump set D/2(xp), jump map g/2(xp), flow set C/2(xp), flow map f/2(xp)
  Integrator System/3 -> j/1
  Integrator System/2 -> t/1
  flow set C/1(inC) -> Integrator System/2
  Integrator System/1 -> state/1, flow map f/1(state), Memory/1
  Integrator System/4 -> jump set D/1(state), jump map g/1(state), flow set C/1(state)
  flow map f/1(dstate) -> Integrator System/1

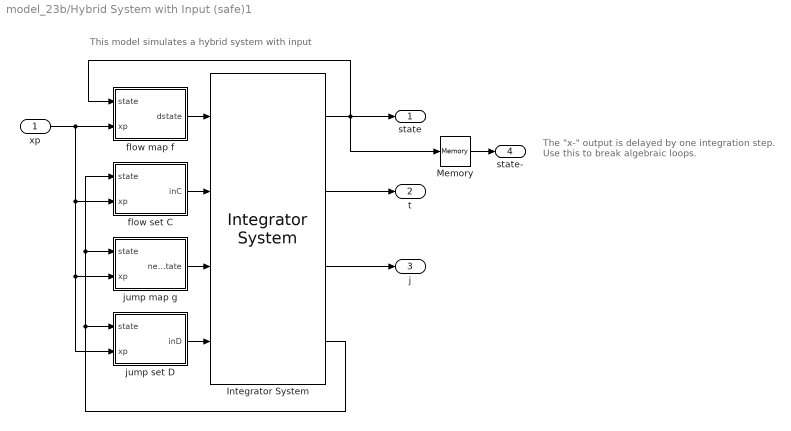
== system model_23b/Hybrid System with Input (safe)1 ==
  note: This model simulates a hybrid system with input
  note: The "x-" output is delayed by one integration step. Use this to break algebraic loops.
  xp : Inport  PortDimensions=input_dim
  Integrator System : HyEQ_Library/Other/Integrator System  Priority=2  T=T  J=J  x0=x0  rule=rule
      link override ICx: Value=xc_0
      link override ICx0: Value=[0; 0; xc_0(:)]
      settings: SourceProductName=Hybrid Equations Toolbox
  Memory : Memory  InitialCondition=x0
  flow map f : MATLAB Function  TreatAsAtomicUnit=on
  flow set C : MATLAB Function  TreatAsAtomicUnit=on
  jump map g : MATLAB Function  TreatAsAtomicUnit=on
  jump set D : MATLAB Function  TreatAsAtomicUnit=on
  state : Outport  PortDimensions=state_dim
  t : Outport  Port=2  PortDimensions=1
  j : Outport  Port=3  PortDimensions=1
  state- : Outport  Port=4  PortDimensions=state_dim
  wires:
  Memory/1 -> state-/1
  jump map g/1(nextstate) -> Integrator System/3
  jump set D/1(inD) -> Integrator System/4
  xp/1 -> jump set D/2(xp), jump map g/2(xp), flow set C/2(xp), flow map f/2(xp)
  Integrator System/3 -> j/1
  Integrator System/2 -> t/1
  flow set C/1(inC) -> Integrator System/2
  Integrator System/1 -> state/1, flow map f/1(state), Memory/1
  Integrator System/4 -> jump set D/1(state), jump map g/1(state), flow set C/1(state)
  flow map f/1(dstate) -> Integrator System/1

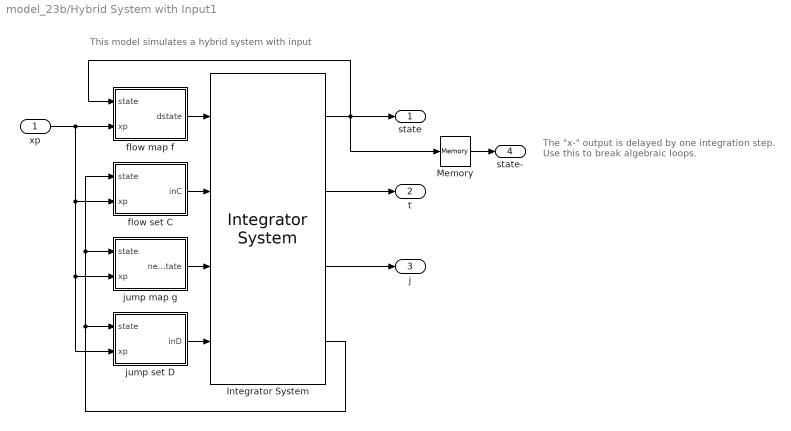
== system model_23b/Hybrid System with Input1 ==
  note: This model simulates a hybrid system with input
  note: The "x-" output is delayed by one integration step. Use this to break algebraic loops.
  xp : Inport  PortDimensions=input_dim
  Integrator System : HyEQ_Library/Other/Integrator System  Priority=2  T=T  J=J  x0=x0  rule=rule
      link override ICx: Value=[xc_0;cal_V0_ini]
      link override ICx0: Value=[0; 0; xc_0;cal_V0_ini]
      settings: SourceProductName=Hybrid Equations Toolbox
  Memory : Memory  InitialCondition=x0
  flow map f : MATLAB Function  TreatAsAtomicUnit=on
  flow set C : MATLAB Function  TreatAsAtomicUnit=on
  jump map g : MATLAB Function  TreatAsAtomicUnit=on
  jump set D : MATLAB Function  TreatAsAtomicUnit=on
  state : Outport  PortDimensions=state_dim
  t : Outport  Port=2  PortDimensions=1
  j : Outport  Port=3  PortDimensions=1
  state- : Outport  Port=4  PortDimensions=state_dim
  wires:
  Memory/1 -> state-/1
  jump map g/1(nextstate) -> Integrator System/3
  jump set D/1(inD) -> Integrator System/4
  xp/1 -> jump set D/2(xp), jump map g/2(xp), flow set C/2(xp), flow map f/2(xp)
  Integrator System/3 -> j/1
  Integrator System/2 -> t/1
  flow set C/1(inC) -> Integrator System/2
  Integrator System/1 -> state/1, flow map f/1(state), Memory/1
  Integrator System/4 -> jump set D/1(state), jump map g/1(state), flow set C/1(state)
  flow map f/1(dstate) -> Integrator System/1

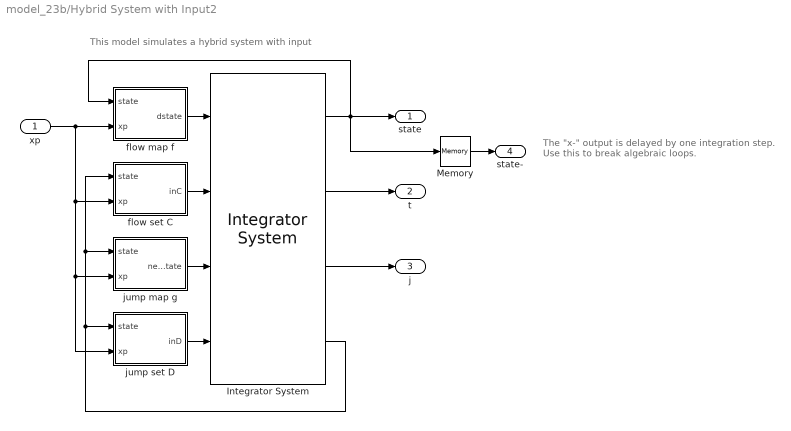
== system model_23b/Hybrid System with Input2 ==
  note: This model simulates a hybrid system with input
  note: The "x-" output is delayed by one integration step. Use this to break algebraic loops.
  xp : Inport  PortDimensions=input_dim
  Integrator System : HyEQ_Library/Other/Integrator System  Priority=2  T=T  J=J  x0=x0  rule=rule
      link override ICx: Value=xc_0
      link override ICx0: Value=[0; 0; xc_0(:)]
      settings: SourceProductName=Hybrid Equations Toolbox
  Memory : Memory  InitialCondition=x0
  flow map f : MATLAB Function  TreatAsAtomicUnit=on
  flow set C : MATLAB Function  TreatAsAtomicUnit=on
  jump map g : MATLAB Function  TreatAsAtomicUnit=on
  jump set D : MATLAB Function  TreatAsAtomicUnit=on
  state : Outport  PortDimensions=state_dim
  t : Outport  Port=2  PortDimensions=1
  j : Outport  Port=3  PortDimensions=1
  state- : Outport  Port=4  PortDimensions=state_dim
  wires:
  Memory/1 -> state-/1
  jump map g/1(nextstate) -> Integrator System/3
  jump set D/1(inD) -> Integrator System/4
  xp/1 -> jump set D/2(xp), jump map g/2(xp), flow set C/2(xp), flow map f/2(xp)
  Integrator System/3 -> j/1
  Integrator System/2 -> t/1
  flow set C/1(inC) -> Integrator System/2
  Integrator System/1 -> state/1, flow map f/1(state), Memory/1
  Integrator System/4 -> jump set D/1(state), jump map g/1(state), flow set C/1(state)
  flow map f/1(dstate) -> Integrator System/1

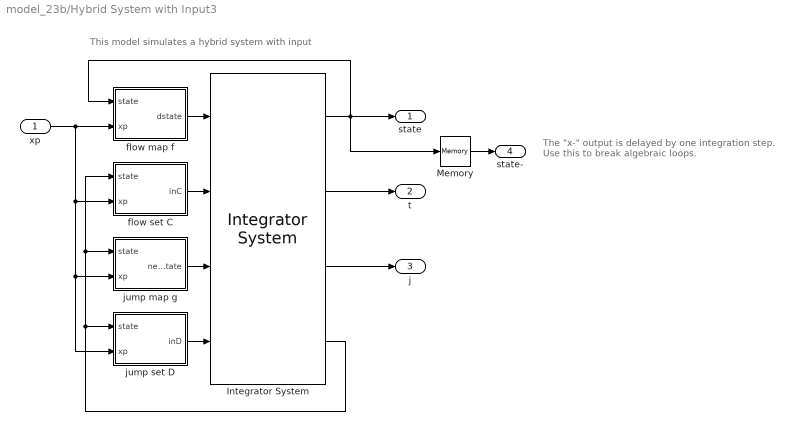
== system model_23b/Hybrid System with Input3 ==
  note: This model simulates a hybrid system with input
  note: The "x-" output is delayed by one integration step. Use this to break algebraic loops.
  xp : Inport  PortDimensions=input_dim
  Integrator System : HyEQ_Library/Other/Integrator System  Priority=2  T=T  J=J  x0=x0  rule=rule
      link override ICx: Value=[xc_0;cal_V0_ini]
      link override ICx0: Value=[0; 0; xc_0;cal_V0_ini]
      settings: SourceProductName=Hybrid Equations Toolbox
  Memory : Memory  InitialCondition=x0
  flow map f : MATLAB Function  TreatAsAtomicUnit=on
  flow set C : MATLAB Function  TreatAsAtomicUnit=on
  jump map g : MATLAB Function  TreatAsAtomicUnit=on
  jump set D : MATLAB Function  TreatAsAtomicUnit=on
  state : Outport  PortDimensions=state_dim
  t : Outport  Port=2  PortDimensions=1
  j : Outport  Port=3  PortDimensions=1
  state- : Outport  Port=4  PortDimensions=state_dim
  wires:
  Memory/1 -> state-/1
  jump map g/1(nextstate) -> Integrator System/3
  jump set D/1(inD) -> Integrator System/4
  xp/1 -> jump set D/2(xp), jump map g/2(xp), flow set C/2(xp), flow map f/2(xp)
  Integrator System/3 -> j/1
  Integrator System/2 -> t/1
  flow set C/1(inC) -> Integrator System/2
  Integrator System/1 -> state/1, flow map f/1(state), Memory/1
  Integrator System/4 -> jump set D/1(state), jump map g/1(state), flow set C/1(state)
  flow map f/1(dstate) -> Integrator System/1

== matlab function model_23b/plant ==
  data: xp input; dxp output; control input; parameters parameter
function dxp = fcn(xp,control,parameters)

dxp=f_p(xp,control,parameters);

end

== matlab function model_23b/Hybrid System with Input (safe)/flow map f ==
  data: state input size=state_dim; xp input size=input_dim; dstate output size=state_dim; parameters parameter
function dstate = f(state, xp, parameters)

dstate=f_flow(state, xp, parameters);

end

== matlab function model_23b/Hybrid System with Input (safe)/flow set C ==
  data: state input size=state_dim; xp input size=input_dim; inC output size=1; parameters parameter
function inC = C(state, xp, parameters)
   [inC,~]=fcn_decide(state,xp,parameters);
end

== matlab function model_23b/Hybrid System with Input (safe)/jump map g ==
  data: state input size=state_dim; xp input size=input_dim; nextstate output size=state_dim; parameters parameter
function nextstate = g(state, xp, parameters)

nextstate=f_jump(state, xp, parameters);

end

== matlab function model_23b/Hybrid System with Input (safe)/jump set D ==
  data: state input size=state_dim; xp input size=input_dim; inD output size=1; parameters parameter
function inD = D(state, xp, parameters)
   [~,inD]=fcn_decide(state,xp,parameters);
end

== matlab function model_23b/Hybrid System with Input1/flow set C ==
  data: state input size=state_dim; xp input size=input_dim; inC output size=1; parameters parameter
function inC = C(state, xp, parameters)

    xc=state(1:3);

   [inC,~]=fcn_decide(xc,xp,parameters);
end

== matlab function model_23b/Hybrid System with Input1/jump map g ==
  data: state input size=state_dim; xp input size=input_dim; nextstate output size=state_dim; parameters parameter
function nextstate = g(state, xp, parameters)

delta=parameters.delta;

xc=state(1:3);
cal_V0=state(4);


nextxc=f_jump(state, xp, parameters);
cal_nextV0=cal_V0-delta;

nextstate=[nextxc;cal_nextV0];

end

== matlab function model_23b/Hybrid System with Input1/jump set D ==
  data: state input size=state_dim; xp input size=input_dim; inD output size=1; parameters parameter
function inD = D(state, xp, parameters)

xc=state(1:3);
   [~,inD]=fcn_decide(xc,xp,parameters);
end

== matlab function model_23b/output eqn of H (safe) ==
  data: xp input; control output; xc input; parameters parameter
function control = fcn(xp,xc,parameters)

x0=[xp;xc];

control=kappa_2(x0,parameters);

end

== matlab function model_23b/plant1 ==
  data: xp input; dxp output; control input; parameters parameter
function dxp = fcn(xp,control,parameters)

dxp=f_p(xp,control,parameters);

end

== matlab function model_23b/MATLAB Function2 ==
  data: xp input; value_a output; xc input; parameters parameter
function value_a = fcn(xp,xc,parameters)

x0=[xp;xc];

value_a=a(x0,parameters);

end

== matlab function model_23b/output eqn of H ==
  data: xp input; control output; xc input; parameters parameter
function control = fcn(xp,xc,parameters)

x0=[xp;xc];

control=kappa_0(x0,parameters);

end

== matlab function model_23b/MATLAB Function3 ==
  data: xp input; value_vartheta1 output; xc input; parameters parameter
function value_vartheta1 = fcn(xp,xc,parameters)

x0=[xp;xc];

value_vartheta1=vartheta1(x0,parameters);

end

== matlab function model_23b/MATLAB Function4 ==
  data: xp input; value_a output; xc input; parameters parameter
function value_a = fcn(xp,xc,parameters)

x0=[xp;xc];

value_a=a(x0,parameters);

end

== matlab function model_23b/MATLAB Function5 ==
  data: xp input; value_vartheta1 output; xc input; parameters parameter
function value_vartheta1 = fcn(xp,xc,parameters)

x0=[xp;xc];

value_vartheta1=vartheta1(x0,parameters);

end

== matlab function model_23b/MATLAB Function6 ==
  data: u input; y output
function y = fcn(u)

y = log(u+eps);

== matlab function model_23b/Lya2 ==
  data: xp input; V0 output; xc input; parameters parameter
function V0 = fcn(xp,xc,parameters)

x0=[xp;xc];

V0=fcn_V0(x0,parameters);

end

== matlab function model_23b/MATLAB Function7 ==
  data: u input; y output
function y = fcn(u)

y = log(u+eps);

== matlab function model_23b/MATLAB Function1 ==
  data: xp input; xc input; min_Lya output; parameters parameter
function min_Lya = fcn(xp,xc,parameters)

%%%
chi=xc(1:2);
% theta=state(3);

%%%
x0_0=[xp;chi;0];%theta=0
x0_1=[xp;chi;1];%theta=1
V0_0=fcn_V0(x0_0,parameters);%theta=0
V0_1=fcn_V0(x0_1,parameters);%theta=1

min_Lya=min(V0_0,V0_1);

end

== matlab function model_23b/Hybrid System with Input (safe)1/flow map f ==
  data: state input size=state_dim; xp input size=input_dim; dstate output size=state_dim; parameters parameter
function dstate = f(state, xp, parameters)

dstate=f_flow(state, xp, parameters);

end

== matlab function model_23b/Hybrid System with Input (safe)1/flow set C ==
  data: state input size=state_dim; xp input size=input_dim; inC output size=1; parameters parameter
function inC = C(state, xp, parameters)
   inC=1;
end

== matlab function model_23b/Hybrid System with Input (safe)1/jump map g ==
  data: state input size=state_dim; xp input size=input_dim; nextstate output size=state_dim; parameters parameter
function nextstate = g(state, xp, parameters)

nextstate=f_jump(state, xp, parameters);

end

== matlab function model_23b/Hybrid System with Input (safe)1/jump set D ==
  data: state input size=state_dim; xp input size=input_dim; inD output size=1; parameters parameter
function inD = D(state, xp, parameters)
   inD=0;
end

== matlab function model_23b/Lya ==
  data: xp input; V0 output; xc input; parameters parameter
function V0 = fcn(xp,xc,parameters)

x0=[xp;xc];

V0=fcn_V0(x0,parameters);

end

== matlab function model_23b/Lya1 ==
  data: xp input; V0 output; xc input; parameters parameter
function V0 = fcn(xp,xc,parameters)

x0=[xp;xc];

V0=fcn_V0(x0,parameters);

end

== matlab function model_23b/MATLAB Function10 ==
  data: xp input; value_vartheta1 output; xc input; parameters parameter
function value_vartheta1 = fcn(xp,xc,parameters)

x0=[xp;xc];

value_vartheta1=vartheta1(x0,parameters);

end

== matlab function model_23b/MATLAB Function11 ==
  data: u input; y output
function y = fcn(u)

y = log(u+eps);

== matlab function model_23b/MATLAB Function8 ==
  data: xp input; xc input; min_Lya output; parameters parameter
function min_Lya = fcn(xp,xc,parameters)

%%%
chi=xc(1:2);
% theta=state(3);

%%%
x0_0=[xp;chi;0];%theta=0
x0_1=[xp;chi;1];%theta=1
V0_0=fcn_V0(x0_0,parameters);%theta=0
V0_1=fcn_V0(x0_1,parameters);%theta=1

min_Lya=min(V0_0,V0_1);

end
